simulink model "EV_Blackstart_Sim"  (R2023b)
settings: Solver=ode45  StartTime=0.0  StopTime=600  RelTol=1e-3
settings Model: Creator=DELL  LastModifiedBy=DELL

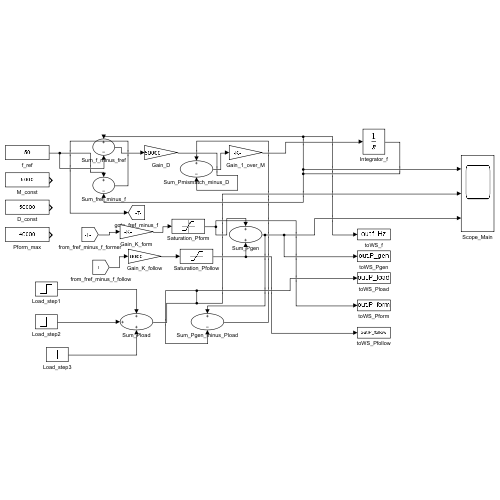
[thumbnail: Simulink's stored preview of the top-level diagram]
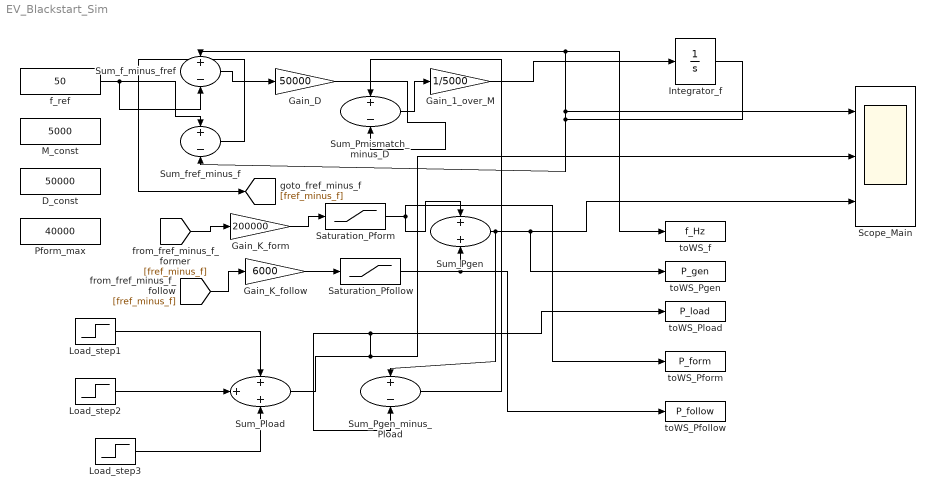
== system EV_Blackstart_Sim ==
  D_const : Constant  Value=50000
  Gain_1_over_M : Gain  Gain=1/5000
  Gain_D : Gain  Gain=50000
  Gain_K_follow : Gain  Gain=6000
  Gain_K_form : Gain  Gain=200000
  Integrator_f : Integrator  InitialCondition=50
  Load_step1 : Step  Time=30  After=100000  SampleTime=0
  Load_step2 : Step  Time=120  After=200000  SampleTime=0
  Load_step3 : Step  Time=240  After=250000  SampleTime=0
  M_const : Constant  Value=5000
  Pform_max : Constant  Value=40000
  Saturation_Pfollow : Saturate  UpperLimit=200000  LowerLimit=0
  Saturation_Pform : Saturate  UpperLimit=40000  LowerLimit=0
  Scope_Main : Scope  NumInputPorts=3
  Sum_Pgen : Sum
  Sum_Pgen_minus_Pload : Sum  Inputs=+-
  Sum_Pload : Sum  Inputs=+++
  Sum_Pmismatch_minus_D : Sum  Inputs=+-
  Sum_f_minus_fref : Sum  Inputs=+-
  Sum_fref_minus_f : Sum  Inputs=+-
  f_ref : Constant  Value=50
  toWS_Pfollow : ToWorkspace  VariableName=P_follow  SaveFormat=Structure With Time  SampleTime=-1
  toWS_Pform : ToWorkspace  VariableName=P_form  SaveFormat=Structure With Time  SampleTime=-1
  toWS_Pgen : ToWorkspace  VariableName=P_gen  SaveFormat=Structure With Time  SampleTime=-1
  toWS_Pload : ToWorkspace  VariableName=P_load  SaveFormat=Structure With Time  SampleTime=-1
  toWS_f : ToWorkspace  VariableName=f_Hz  SaveFormat=Structure With Time  SampleTime=-1
  wires:
  Integrator_f/1 -> Sum_f_minus_fref/1, toWS_f/1, Scope_Main/1, Sum_fref_minus_f/2
  f_ref/1 -> Sum_f_minus_fref/2, Sum_fref_minus_f/1
  Sum_f_minus_fref/1 -> Gain_D/1
  Sum_fref_minus_f/1 -> [fref_minus_f]
  [fref_minus_f] -> Gain_K_form/1
  Gain_K_form/1 -> Saturation_Pform/1
  [fref_minus_f] -> Gain_K_follow/1
  Gain_K_follow/1 -> Saturation_Pfollow/1
  Saturation_Pform/1 -> Sum_Pgen/1, toWS_Pform/1
  Saturation_Pfollow/1 -> Sum_Pgen/2, toWS_Pfollow/1
  Load_step1/1 -> Sum_Pload/1
  Load_step2/1 -> Sum_Pload/2
  Load_step3/1 -> Sum_Pload/3
  Sum_Pgen/1 -> Scope_Main/3, toWS_Pgen/1, Sum_Pgen_minus_Pload/1
  Sum_Pload/1 -> Sum_Pgen_minus_Pload/2, toWS_Pload/1, Scope_Main/2
  Sum_Pgen_minus_Pload/1 -> Sum_Pmismatch_minus_D/1
  Gain_D/1 -> Sum_Pmismatch_minus_D/2
  Sum_Pmismatch_minus_D/1 -> Gain_1_over_M/1
  Gain_1_over_M/1 -> Integrator_f/1
